simulink model "XTHERM05_reference"  (R2025a)
settings: Solver=daessc  StartTime=0  StopTime=240  MaxStep=1  RelTol=1e-3  AbsTol=1e-3
undefined symbols (not defined in the file): battery_builder_rtmsupport, charge_current_A, charge_step_fraction, charge_step_time_s, coolant_inlet_temperature_K, gcbh, initial_battery_temperature_K
libraries: BatteryPack96S3P_lib x12, fl_lib x8, nesl_utility x5, BatteryCurrentManagement x1, coolingPlateThermal_lib x1
(part 1 of 3)
settings Model: Creator=abirdas  LastModifiedBy=SimuVerity Contributors
settings SolverCC: AutoScaleAbsTol=off
settings SimscapeCC: SimscapeLogType=all  SimscapeLogName=SimlogBattery  SimscapeLogLimitData=off  SimscapeCompileComponentReuse=on
settings ExplorerConfigSet: SimMechanicsOpenEditorOnUpdate=off

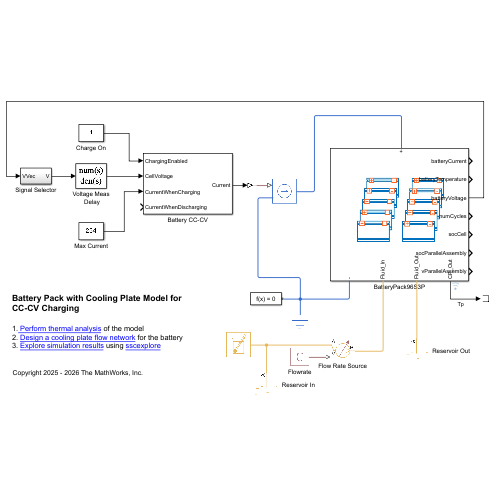
[thumbnail: Simulink's stored preview of the top-level diagram]
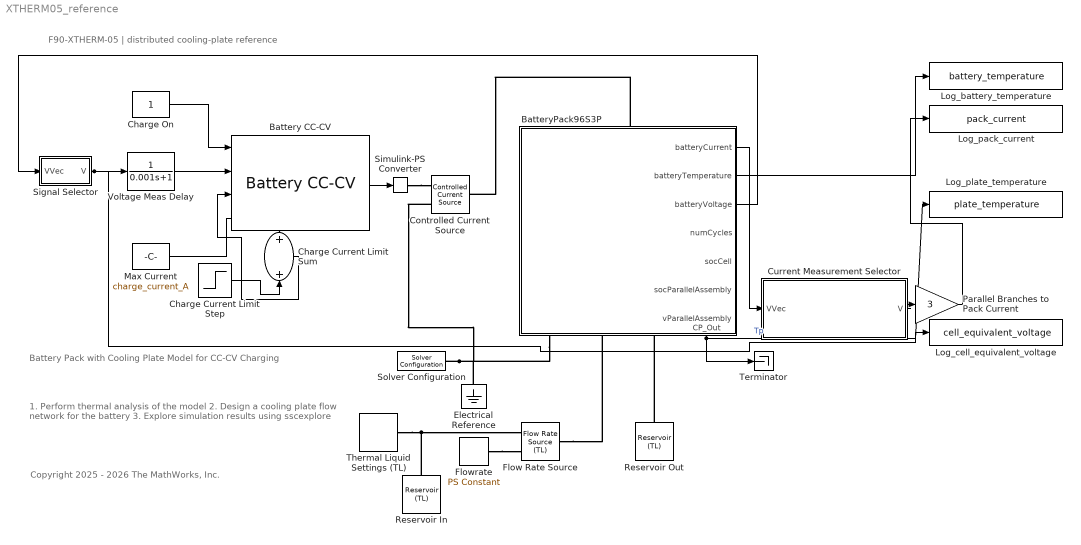
== system XTHERM05_reference ==
  note: 1. Perform thermal analysis of the model
      | 2. Design a cooling plate flow network for the battery
      | 3. Explore simulation results using sscexplore
  note: Copyright 2025 - 2026 The MathWorks, Inc.
  note: Battery Pack with Cooling Plate Model for CC-CV Charging
  note: F90-XTHERM-05 | distributed cooling-plate reference
  Battery CC-CV : BatteryCurrentManagement/Battery CC-CV  MinMaxFlag=off  MaxCellVoltage=max_cell_voltage_V  Kp=100  Ki=1  Kaw=1  Kt=1  Ts=1
      settings: LibrarySourceBlock=batt_sl_lib/Current Management/Battery CC-CV
  BatteryPack96S3P : Subsystem  LoadFcn=battery_builder_rtmsupport('loadfcn',gcbh);
      settings: CopyFcn=battery_builder_rtmsupport('copyfcn',gcbh);  PreCopyFcn=battery_builder_rtmsupport('precopyfcn',gcbh);  PreDeleteFcn=battery_builder_rtmsupport('predeletefcn',gcbh);  PortSchema="{\"entries\":[{\"content\":{\"sides\":[{\"content\":{\"connectorIds\":[\"LConn1\"]},\"type\":\"ConnectorPlacement.EquallySpacedRectSide\",\"uuid\":\"f2fadea4-e63e-44ff-a05d-5cbabbfa18f3\"},{\"content\":{\"connectorIds\":[\"RConn1\",\"RConn2\",\"RConn3\",\"Out1\"],\"side\":\"RIGHT\"},\"type\":\"ConnectorPlacement.EquallySpacedRectSide\",\"uuid\":\"922c0eb8-6335-439b-a096-ecac4f67b25b\"},{\"content\":{\"side\":\"TOP\"},\"type\":\"ConnectorPlacement.EquallySpacedRectSide\",\"uuid\":\"a4ac09f9-1b8b-4b5a-a998-1dae1de64a0b\"},{\"content\":{\"connectorIds\":[\"Out2\",\"Out3\",\"Out4\",\"Out5\",\"Out6\",\"Out7\",\"Out8\"],\"side\":\"BOTTOM\"},\"type\":\"ConnectorPlacement.EquallySpacedRectSide\",\"uuid\":\"64bbb320-f65b-462a-a8f2-7dda0291aa0b\"}]},\"type\":\"ConnectorPlacement.EquallySpacedConnector\",\"uuid\":\"78c9e32e-0392-43f3-93f6-199d4a6b3441\"}],\"packageUris\":[\"http://schema.mathworks.com/mf0/Connector/R2020b\"],\"version\":\"1.0\"}"
      mask Display: image('$imagefile')
  Charge Current Limit Step : Step  Time=charge_step_time_s  After=charge_current_A*charge_step_fraction  SampleTime=0
  Charge Current Limit Sum : Sum
  Charge On : Constant
  Controlled Current Source : fl_lib/Electrical/Electrical Sources/Controlled Current Source
  Current Measurement Selector : Subsystem
  Electrical Reference : fl_lib/Electrical/Electrical Elements/Electrical Reference
  Flow Rate Source : fl_lib/Thermal Liquid/Sources/Flow Rate Source (TL)  source_type=foundation.enum.constant_controlled.controlled  flow_type=foundation.enum.mass_volumetric_flow.volumetric  mass_flow=0 kg/s  volumetric_flow=0 m^3/s  power_spec=foundation.enum.power_spec.isentropic  area=0.01 m^2
      settings: InternalSimscapePortConfiguration="{\"Bottom\":[],\"Left\":[{\"id\":\"A\",\"label\":\"A\",\"type\":\"foundation.thermal_liquid.thermal_liquid\"},{\"id\":\"V\",\"label\":\"V\",\"type\":\"input\"}],\"Right\":[{\"id\":\"B\",\"label\":\"B\",\"type\":\"foundation.thermal_liquid.thermal_liquid\"}],\"Top\":[]}"
  Flowrate : fl_lib/Physical Signals/Sources/PS Constant  constant=coolant_flow_lpm lpm
  Log_battery_temperature : ToWorkspace  VariableName=battery_temperature  SaveFormat=Timeseries  SampleTime=-1
  Log_cell_equivalent_voltage : ToWorkspace  VariableName=cell_equivalent_voltage  SaveFormat=Timeseries  SampleTime=-1
  Log_pack_current : ToWorkspace  VariableName=pack_current  SaveFormat=Timeseries  SampleTime=-1
  Log_plate_temperature : ToWorkspace  VariableName=plate_temperature  SaveFormat=Timeseries  SampleTime=-1
  Max Current : Constant  Value=charge_current_A
  Parallel Branches to Pack Current : Gain  Gain=3
  Reservoir In : fl_lib/Thermal Liquid/Elements/Reservoir (TL)  pressure_spec=foundation.enum.pressure_spec.atmospheric  reservoir_pressure=0.101325 MPa  reservoir_temperature=coolant_inlet_temperature_K K  area=0.01 m^2
  Reservoir Out : fl_lib/Thermal Liquid/Elements/Reservoir (TL)  pressure_spec=foundation.enum.pressure_spec.atmospheric  reservoir_pressure=0.101325 MPa  reservoir_temperature=coolant_inlet_temperature_K K  area=0.01 m^2
  Signal Selector : Subsystem
  Simulink-PS Converter : nesl_utility/Simulink-PS Converter  PhysicalDomain=network_engine_domain  SubClassName=ps_input  LeftPortType=input  RightPortType=output  PseudoPeriodic=off  Frequencies=[]  NoiseDistribution=none  NoiseParameters=[]  Unit=1  AffineConversion=off  FilteringAndDerivatives=provide  SimscapeFilterOrder=1  InputFilterTimeConstant=0.001  UdotUserProvided=0
  Solver Configuration : nesl_utility/Solver Configuration  PhysicalDomain=network_engine_domain  SubClassName=solver  LeftPortType=input  RightPortType=generic  Tones=[]  Harmonics=[]  SimulateNoise=off  Profile=off  UseLocalSampling=off  EnableSwitchedLinearOptims=on  FrequencyDomain=off  UseCCode=off  RelTol=0.001  AbsTol=0.001  MinStep=1e-09  ToWorkspace=off  RevertToSquareIcSolve=off  NumHomotopyIterations=100  PhasorMode=off  PhasorModeNumHarmonics=1  ConsistencySolver=NEWTON_XTOL_AFTER_FTOL  IndexReductionMethod=DerivativeReplacement  DoDC=off  ResidualTolerance=1e-09  ConsistencyTolSource=GLOBAL  ConsistencyAbsTol=0.001  ConsistencyRelTol=0.001  ConsistencyTolFactor=0.001  UseLocalSolver=off  LocalSolverChoice=NE_BACKWARD_EULER_ADVANCER  ResolveIndetEquations=on  FunctionEvalNumThread=1  LocalSolverSampleTime=0.001  DoFixedCost=off  MaxNonlinIter=3  MaxModeIter=2  ComputeImpulses=off  ImpulseIterations=2  LinearAlgebra=auto  LinearAlgebraNumThread=0  EquationFormulation=NE_TIME_EF  DelaysMemoryBudget=1024  AutomaticFiltering=on  FilteringTimeConstant=0.001  PartitionStorageMethod=AS_NEEDED  PartitionMemoryBudget=1024  PartitionMethod=ROBUST  MultibodyUseLocalSolver=off  MultibodyLocalSolverChoice=ODE1  MultibodyLocalSolverSampleTime=0.001
  Terminator : Terminator
  Thermal Liquid Settings (TL) : fl_lib/Thermal Liquid/Utilities/Thermal Liquid Settings (TL)  table_dimensions=foundation.enum.table_dimensions_TL.two_dimensional  T_TLU=[273.1600 : 10 : 373.16]' K  p_TLU=[0.01, 0.1, 5 : 5 : 50] MPa  p_atm=0.101325 MPa  pT_region_flag=foundation.enum.pT_region_TL.min_max  T_min=273.16 K  T_max=373.16 K  p_min=0.01 MPa  p_max=50 MPa  T_min_1D=273.16 K  T_max_1D=373.16 K  p_min_1D=0.01 MPa  p_max_1D=50 MPa  pT_validity_TLU=[1, 1, 1, 1, 1, 1, 1, 1, 1, 1, 1, 1; 1, 1, 1, 1, 1, 1, 1, 1, 1, 1, 1, 1; 1, 1, 1, 1, 1, 1, 1, 1, 1, 1, 1, 1; 1, 1, 1, 1, 1, 1, 1, 1, 1, 1, 1, 1; 1, 1, 1, 1, 1, 1, 1, 1, 1, 1, 1, 1; 0, 1, 1, 1, 1, 1, 1, 1, 1, 1, 1, 1; 0, 1, 1, 1, 1, 1, 1, 1, 1, 1, 1, 1; 0, 1, 1, 1, 1, 1, 1, 1, 1, 1, 1, 1; 0, 1, 1, 1, 1, 1, 1, 1, 1, 1, 1, 1; 0, 1, 1, 1, 1, 1, 1, 1, 1, 1, 1, 1; 0, 0, 1, 1, 1, 1, 1, 1, 1, 1, 1, 1]  properties_range_check=simscape.enum.assert.action.error  rho_parameterization_2D=foundation.enum.rho_parameterization_2D.rho_beta_alpha  rho_parameterization_1D=foundation.enum.rho_parameterization_1D.rho_vector  rho_TLU=[999.7973, 999.8431, 1002.3216, 1004.8218, 1007.293, 1009.7358, 1012.1506, 1014.5379, 1016.8979, 1019.2311, 1021.538, 1023.8188; 999.6579, 999.7009, 1002.0303, 1004.382, 1006.7084, 1009.0101, 1011.2874, 1013.5407, 1015.7703, 1017.9766, 1020.1599, 1022.3206; 998.1632, 998.2045, 1000.4375, 1002.6924, 1004.9239, 1007.1324, 1009.3183, 1011.4819, 1013.6236, 1015.7438, 1017.8428, 1019.921; 995.6057, 995.6458, 997.8186, 1000.0128, 1002.1841, 1004.3332, 1006.4603, 1008.566, 1010.6505, 1012.7144, 1014.758, 1016.7815; 992.1724, 992.2119, 994.3513, 996.5113, 998.6484, 1000.7633, 1002.8563, 1004.928, 1006.9788, 1009.009, 1011.0192, 1013.0097; 988.02, 988.0299, 990.1568, 992.3035, 994.4268, 996.5273, 998.6056, 1000.6622, 1002.6976, 1004.7123, 1006.7067, 1008.6813; 983.18, 983.1901, 985.3217, 987.4721, 989.5983, 991.7008, 993.7803, 995.8374, 997.8726, 999.8864, 1001.8795, 1003.8522; 977.75, 977.7583, 979.9094, 982.0783, 984.2216, 986.34, 988.4343, 990.505, 992.5529, 994.5786, 996.5825, 998.5654; 971.77, 971.7836, 973.9673, 976.1678, 978.3409, 980.4876, 982.6087, 984.7049, 986.7768, 988.8254, 990.8511, 992.8545; 965.26, 965.3023, 967.5311, 969.7753, 971.9901, 974.1764, 976.3354, 978.4676, 980.5741, 982.6556, 984.7129, 986.7465; 958.62, 958.6315, 960.627, 962.9267, 965.1944, 967.4314, 969.6387, 971.8173, 973.9681, 976.0921, 978.19, 980.2628] kg/m^3  beta_TLU=[1.9649, 1.9654, 1.9929, 2.0213, 2.0499, 2.0787, 2.1078, 2.1372, 2.1668, 2.1966, 2.2268, 2.2572; 2.0913, 2.0918, 2.1191, 2.1471, 2.1752, 2.2036, 2.2322, 2.261, 2.2899, 2.3191, 2.3485, 2.3781; 2.1786, 2.1791, 2.2067, 2.235, 2.2634, 2.2919, 2.3206, 2.3494, 2.3784, 2.4075, 2.4367, 2.4661; 2.2332, 2.2337, 2.2619, 2.2908, 2.3197, 2.3487, 2.3778, 2.407, 2.4363, 2.4657, 2.4951, 2.5246; 2.26, 2.2605, 2.2895, 2.3191, 2.3487, 2.3784, 2.4081, 2.4378, 2.4675, 2.4973, 2.5272, 2.5571; 2.2638, 2.2638, 2.2936, 2.324, 2.3544, 2.3848, 2.4151, 2.4455, 2.4758, 2.5062, 2.5365, 2.5669; 2.2472, 2.2472, 2.2779, 2.3092, 2.3403, 2.3715, 2.4025, 2.4336, 2.4646, 2.4955, 2.5264, 2.5573; 2.214, 2.214, 2.2455, 2.2776, 2.3096, 2.3415, 2.3733, 2.405, 2.4367, 2.4683, 2.4998, 2.5313; 2.1668, 2.1668, 2.1992, 2.2321, 2.2649, 2.2976, 2.3301, 2.3626, 2.3949, 2.4272, 2.4593, 2.4914; 2.1081, 2.1081, 2.1413, 2.175, 2.2086, 2.2421, 2.2754, 2.3085, 2.3415, 2.3744, 2.4072, 2.4399; 2.0494, 2.0494, 2.0739, 2.1084, 2.1428, 2.177, 2.211, 2.2449, 2.2786, 2.3121, 2.3455, 2.3788] GPa  alpha_TLU=1e-4 * [-.679, -.676, -.49, -.307, -.13, .041, .206, .365, .519, .668, .811, .949; .878, .881, .998, 1.114, 1.227, 1.337, 1.445, 1.549, 1.651, 1.75, 1.846, 1.939; 2.068, 2.069, 2.141, 2.213, 2.283, 2.352, 2.42, 2.486, 2.551, 2.614, 2.676, 2.736; 3.034, 3.035, 3.074, 3.113, 3.152, 3.191, 3.229, 3.267, 3.305, 3.341, 3.377, 3.413; 3.855, 3.856, 3.87, 3.884, 3.899, 3.914, 3.93, 3.946, 3.961, 3.977, 3.993, 4.009; 4.578, 4.578, 4.572, 4.566, 4.562, 4.558, 4.555, 4.552, 4.55, 4.549, 4.548, 4.547; 5.233, 5.233, 5.209, 5.186, 5.165, 5.144, 5.125, 5.107, 5.09, 5.074, 5.059, 5.045; 5.84, 5.84, 5.801, 5.762, 5.725, 5.691, 5.657, 5.625, 5.595, 5.566, 5.538, 5.512; 6.414, 6.414, 6.36, 6.307, 6.256, 6.208, 6.161, 6.117, 6.074, 6.033, 5.994, 5.956; 6.967, 6.967, 6.898, 6.831, 6.766, 6.705, 6.646, 6.589, 6.535, 6.482, 6.432, 6.384; 7.519, 7.519, 7.423, 7.342, 7.264, 7.189, 7.118, 7.049, 6.983, 6.92, 6.859, 6.8] 1/K  rho_TLU_2=[999.7973, 999.8431, 1002.3216, 1004.8218, 1007.293, 1009.7358, 1012.1506, 1014.5379, 1016.8979, 1019.2311, 1021.538, 1023.8188; 999.6579, 999.7009, 1002.0303, 1004.382, 1006.7084, 1009.0101, 1011.2874, 1013.5407, 1015.7703, 1017.9766, 1020.1599, 1022.3206; 998.1632, 998.2045, 1000.4375, 1002.6924, 1004.9239, 1007.1324, 1009.3183, 1011.4819, 1013.6236, 1015.7438, 1017.8428, 1019.921; 995.6057, 995.6458, 997.81864, 1000.0128, 1002.1841, 1004.3332, 1006.4603, 1008.566, 1010.6505, 1012.7144, 1014.758, 1016.7815; 992.1724, 992.2119, 994.3513, 996.5113, 998.6484, 1000.7633, 1002.8563, 1004.928, 1006.9788, 1009.009, 1011.0192, 1013.0097; 988.02, 988.0299, 990.1568, 992.3035, 994.4268, 996.5273, 998.6056, 1000.6622, 1002.6976, 1004.7123, 1006.7067, 1008.6813; 983.18, 983.1901, 985.3217, 987.4721, 989.5983, 991.7008, 993.7803, 995.8374, 997.8726, 999.8864, 1001.8795, 1003.8522; 977.75, 977.7583, 979.9094, 982.0783, 984.2216, 986.34, 988.4343, 990.505, 992.5529, 994.5786, 996.5825, 998.5654; 971.77, 971.7836, 973.9673, 976.1678, 978.3409, 980.4876, 982.6087, 984.7049, 986.7768, 988.8254, 990.8511, 992.8545; 965.26, 965.3023, 967.5311, 969.7753, 971.9901, 974.1764, 976.3354, 978.4676, 980.5741, 982.6556, 984.7129, 986.7465; 958.62, 958.6315, 960.627, 962.9267, 965.1944, 967.4314, 969.6387, 971.8173, 973.9681, 976.0921, 978.19, 980.2628] kg/m^3  rho_ref_3=998.21 kg/m^3  T_ref_3=293.16 K  p_ref_3=0.101325 MPa  beta_const_3=2.1791 GPa  alpha_const_3=2.0691e-4 1/K  rho_TLU_4=[999.84; 999.7; 998.2; 995.65; 992.21; 988.03; 983.19; 977.76; 971.78; 965.3; 958.8] kg/m^3  beta_const_4=2.1791 GPa  p_ref_4=0.101325 MPa  rho_ref_5=998.21 kg/m^3  T_ref_5=293.16 K  p_ref_5=0.101325 MPa  beta_const_5=2.1791 GPa  alpha_const_5=2.0691e-4 1/K  u_parameterization_2D=foundation.enum.u_parameterization_2D.u_cp  u_parameterization_1D=foundation.enum.u_parameterization_1D.u  u_TLU=[.0002, .0018, .086, .1588, .219, .267, .3034, .3288, .3436, .3483, .3435, .3294; 42.062, 42.06, 41.935, 41.804, 41.668, 41.527, 41.382, 41.233, 41.081, 40.924, 40.763, 40.599; 83.953, 83.948, 83.651, 83.349, 83.049, 82.749, 82.451, 82.153, 81.856, 81.56, 81.265, 80.971; 125.77, 125.76, 125.31, 124.86, 124.41, 123.97, 123.53, 123.1, 122.68, 122.25, 121.84, 121.42; 167.57, 167.56, 166.96, 166.37, 165.79, 165.21, 164.65, 164.09, 163.54, 163, 162.46, 161.94; 209.36, 209.36, 208.63, 207.9, 207.19, 206.48, 205.79, 205.11, 204.45, 203.79, 203.14, 202.5; 251.19, 251.19, 250.33, 249.47, 248.62, 247.79, 246.98, 246.18, 245.39, 244.62, 243.86, 243.12; 293.06, 293.06, 292.07, 291.07, 290.1, 289.14, 288.2, 287.28, 286.38, 285.49, 284.62, 283.77; 334.99, 334.99, 333.86, 332.73, 331.63, 330.54, 329.48, 328.44, 327.41, 326.41, 325.43, 324.46; 377, 377, 375.73, 374.46, 373.22, 372, 370.81, 369.64, 368.5, 367.38, 366.27, 365.19; 419.01, 419.01, 417.69, 416.27, 414.89, 413.54, 412.21, 410.91, 409.64, 408.4, 407.17, 405.98] kJ/kg  cp_TLU=[4.2199, 4.2194, 4.1957, 4.1726, 4.1508, 4.13, 4.1103, 4.0916, 4.0738, 4.0569, 4.0408, 4.0254; 4.1955, 4.1951, 4.1769, 4.1592, 4.1422, 4.1259, 4.1103, 4.0954, 4.0812, 4.0676, 4.0545, 4.0421; 4.1843, 4.184, 4.169, 4.1543, 4.1401, 4.1264, 4.1133, 4.1007, 4.0885, 4.0768, 4.0656, 4.0548; 4.1801, 4.1798, 4.1667, 4.1538, 4.1413, 4.1293, 4.1177, 4.1064, 4.0956, 4.0851, 4.075, 4.0653; 4.1796, 4.1794, 4.1675, 4.1558, 4.1444, 4.1334, 4.1227, 4.1123, 4.1023, 4.0926, 4.0832, 4.0741; 4.1813, 4.1813, 4.1702, 4.1592, 4.1484, 4.138, 4.1279, 4.1181, 4.1086, 4.0993, 4.0903, 4.0816; 4.185, 4.185, 4.1742, 4.1636, 4.1532, 4.1432, 4.1334, 4.1239, 4.1146, 4.1056, 4.0969, 4.0884; 4.1901, 4.1901, 4.1795, 4.169, 4.1588, 4.1489, 4.1393, 4.1299, 4.1207, 4.1118, 4.1032, 4.0947; 4.1968, 4.1968, 4.1862, 4.1757, 4.1655, 4.1555, 4.1458, 4.1364, 4.1273, 4.1183, 4.1096, 4.1012; 4.2052, 4.2052, 4.1944, 4.1837, 4.1733, 4.1632, 4.1534, 4.1438, 4.1345, 4.1255, 4.1166, 4.108; 4.2136, 4.2136, 4.2045, 4.1935, 4.1828, 4.1724, 4.1623, 4.1524, 4.1429, 4.1335, 4.1245, 4.1157] kJ/(K*kg)  u_TLU_2=[.0002, .0018, .086, .1588, .219, .267, .3034, .3288, .3436, .3483, .3435, .3294; 42.062, 42.06, 41.935, 41.804, 41.668, 41.527, 41.382, 41.233, 41.081, 40.924, 40.763, 40.599; 83.953, 83.948, 83.651, 83.349, 83.049, 82.749, 82.451, 82.153, 81.856, 81.56, 81.265, 80.971; 125.77, 125.76, 125.31, 124.86, 124.41, 123.97, 123.53, 123.1, 122.68, 122.25, 121.84, 121.42; 167.57, 167.56, 166.96, 166.37, 165.79, 165.21, 164.65, 164.09, 163.54, 163, 162.46, 161.94; 209.36, 209.36, 208.63, 207.9, 207.19, 206.48, 205.79, 205.11, 204.45, 203.79, 203.14, 202.5; 251.19, 251.19, 250.33, 249.47, 248.62, 247.79, 246.98, 246.18, 245.39, 244.62, 243.86, 243.12; 293.06, 293.06, 292.07, 291.07, 290.1, 289.14, 288.2, 287.28, 286.38, 285.49, 284.62, 283.77; 334.99, 334.99, 333.86, 332.73, 331.63, 330.54, 329.48, 328.44, 327.41, 326.41, 325.43, 324.46; 377, 377, 375.73, 374.46, 373.22, 372, 370.81, 369.64, 368.5, 367.38, 366.27, 365.19; 419.01, 419.01, 417.69, 416.27, 414.89, 413.54, 412.21, 410.91, 409.64, 408.4, 407.17, 405.98] kJ/kg  cp_TLU_3=[4.2199, 4.2194, 4.1957, 4.1726, 4.1508, 4.13, 4.1103, 4.0916, 4.0738, 4.0569, 4.0408, 4.0254; 4.1955, 4.1951, 4.1769, 4.1592, 4.1422, 4.1259, 4.1103, 4.0954, 4.0812, 4.0676, 4.0545, 4.0421; 4.1843, 4.184, 4.169, 4.1543, 4.1401, 4.1264, 4.1133, 4.1007, 4.0885, 4.0768, 4.0656, 4.0548; 4.1801, 4.1798, 4.1667, 4.1538, 4.1413, 4.1293, 4.1177, 4.1064, 4.0956, 4.0851, 4.075, 4.0653; 4.1796, 4.1794, 4.1675, 4.1558, 4.1444, 4.1334, 4.1227, 4.1123, 4.1023, 4.0926, 4.0832, 4.0741; 4.1813, 4.1813, 4.1702, 4.1592, 4.1484, 4.138, 4.1279, 4.1181, 4.1086, 4.0993, 4.0903, 4.0816; 4.185, 4.185, 4.1742, 4.1636, 4.1532, 4.1432, 4.1334, 4.1239, 4.1146, 4.1056, 4.0969, 4.0884; 4.1901, 4.1901, 4.1795, 4.169, 4.1588, 4.1489, 4.1393, 4.1299, 4.1207, 4.1118, 4.1032, 4.0947; 4.1968, 4.1968, 4.1862, 4.1757, 4.1655, 4.1555, 4.1458, 4.1364, 4.1273, 4.1183, 4.1096, 4.1012; 4.2052, 4.2052, 4.1944, 4.1837, 4.1733, 4.1632, 4.1534, 4.1438, 4.1345, 4.1255, 4.1166, 4.108; 4.2136, 4.2136, 4.2045, 4.1935, 4.1828, 4.1724, 4.1623, 4.1524, 4.1429, 4.1335, 4.1245, 4.1157] kJ/(K*kg)  u_TLU_4=[.0018; 42.06; 83.948; 125.76; 167.56; 209.36; 251.19; 293.06; 334.99; 377; 418.01] kJ/kg  cp_TLU_5=[4.2199; 4.1955; 4.1843; 4.1801; 4.1796; 4.1813; 4.185; 4.1901; 4.1968; 4.2052; 4.2136] kJ/(K*kg)  nu_TLU=[1.7917, 1.7914, 1.7763, 1.7615, 1.7473, 1.7338, 1.7208, 1.7085, 1.6967, 1.6854, 1.6747, 1.6645; 1.3061, 1.3059, 1.2986, 1.2914, 1.2845, 1.2779, 1.2716, 1.2656, 1.2598, 1.2543, 1.2491, 1.2441; 1.0032, 1.0032, .9995, .9959, .9924, .9891, .9859, .9829, .9801, .9774, .9748, .9724; .8006, .8005, .7987, .797, .7953, .7937, .7922, .7908, .7894, .7881, .787, .7859; .6577, .6577, .657, .6562, .6555, .6548, .6543, .6537, .6532, .6528, .6523, .652; .553, .553, .5529, .5527, .5526, .5525, .5524, .5524, .5524, .5524, .5524, .5525; .4739, .4739, .4741, .4743, .4745, .4747, .475, .4753, .4755, .4758, .4762, .4765; .4127, .4127, .4131, .4135, .4139, .4143, .4148, .4152, .4157, .4162, .4167, .4172; .3643, .3643, .3648, .3654, .3659, .3665, .367, .3676, .3682, .3688, .3694, .37; .3254, .3254, .3261, .3267, .3273, .328, .3286, .3293, .3299, .3306, .3312, .3319; .2866, .2866, .2945, .2952, .2959, .2965, .2972, .2979, .2986, .2993, .3, .3007] mm^2/s  nu_TLU_2=[1.7917; 1.3061; 1.0032; .8006; .6577; .553; .4739; .4127; .3643; .3254; .2866] mm^2/s  k_TLU=[561.04, 561.09, 563.8, 566.56, 569.32, 572.08, 574.82, 577.54, 580.24, 582.92, 585.57, 588.18; 580.02, 580.07, 582.45, 584.88, 587.32, 589.75, 592.18, 594.61, 597.02, 599.42, 601.8, 604.16; 598.44, 598.48, 600.73, 603.03, 605.33, 607.64, 609.94, 612.24, 614.54, 616.82, 619.1, 621.36; 615.48, 615.52, 617.73, 620, 622.26, 624.54, 626.81, 629.07, 631.34, 633.6, 635.85, 638.09; 630.6, 630.64, 632.87, 635.15, 637.44, 639.72, 642.01, 644.29, 646.57, 648.84, 651.11, 653.36; 643.61, 643.61, 645.88, 648.21, 650.53, 652.86, 655.18, 657.51, 659.82, 662.14, 664.44, 666.74; 654.39, 654.39, 656.73, 659.12, 661.5, 663.89, 666.27, 668.65, 671.02, 673.38, 675.74, 678.09; 663.13, 663.13, 665.54, 668, 670.46, 672.91, 675.36, 677.8, 680.24, 682.67, 685.09, 687.5; 670.02, 670.02, 672.51, 675.05, 677.59, 680.12, 682.64, 685.16, 687.67, 690.17, 692.66, 695.14; 675.27, 675.27, 677.85, 680.48, 683.11, 685.73, 688.34, 690.94, 693.53, 696.11, 698.68, 701.24; 680.52, 680.52, 681.77, 684.5, 687.22, 689.94, 692.64, 695.34, 698.02, 700.69, 703.35, 706] mW/(K*m)  k_TLU_2=[561.04; 580.02; 598.44; 615.48; 630.6; 643.61; 654.39; 663.13; 670.02; 675.27; 680.52] mW/(K*m)
  Voltage Meas Delay : TransferFcn  Denominator=[0.001 1]
  wires:
  Signal Selector/1(V) -> Voltage Meas Delay/1, Log_cell_equivalent_voltage/1
  Battery CC-CV/1 -> Simulink-PS Converter/1
  Voltage Meas Delay/1 -> Battery CC-CV/2
  Charge On/1 -> Battery CC-CV/1
  BatteryPack96S3P/1(CP_Out) -> Terminator/1, Log_plate_temperature/1  "Tp"
  BatteryPack96S3P/4(batteryVoltage) -> Signal Selector/1(VVec)
  Max Current/1 -> Charge Current Limit Sum/1
  Charge Current Limit Step/1 -> Charge Current Limit Sum/2
  Charge Current Limit Sum/1 -> Battery CC-CV/3
  BatteryPack96S3P/3(batteryTemperature) -> Log_battery_temperature/1
  BatteryPack96S3P/2(batteryCurrent) -> Current Measurement Selector/1(VVec)
  Current Measurement Selector/1(V) -> Parallel Branches to Pack Current/1
  Parallel Branches to Pack Current/1 -> Log_pack_current/1
  connections:
  Thermal Liquid Settings (TL)/RConn1 -- Flow Rate Source/LConn1 -- Reservoir In/LConn1
  Solver Configuration/RConn1 -- BatteryPack96S3P/RConn1 -- Electrical Reference/LConn1 -- Controlled Current Source/RConn2
  Simulink-PS Converter/RConn1 -- Controlled Current Source/RConn1
  BatteryPack96S3P/LConn1 -- Controlled Current Source/LConn1
  Flowrate/RConn1 -- Flow Rate Source/LConn2
  Reservoir Out/LConn1 -- BatteryPack96S3P/RConn3
  Flow Rate Source/RConn1 -- BatteryPack96S3P/RConn2

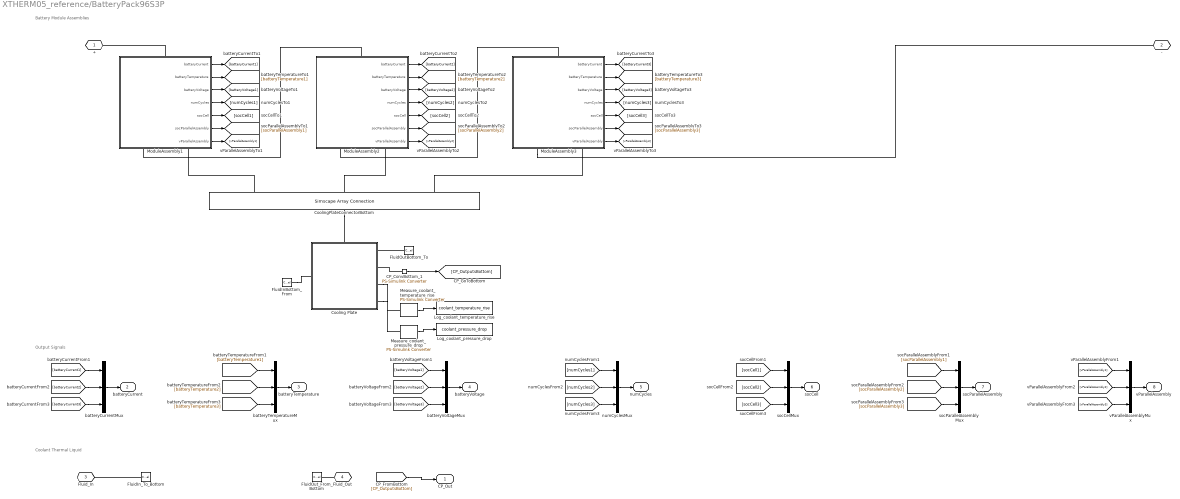
== system XTHERM05_reference/BatteryPack96S3P ==
  note: Battery Module Assemblies
  note: Output Signals
  note: Coolant Thermal Liquid
  CP_ConvBottom_1 : nesl_utility/PS-Simulink Converter  PhysicalDomain=network_engine_domain  SubClassName=ps_output  LeftPortType=input  RightPortType=output  PseudoPeriodic=off  Frequencies=[]  VectorFormat=inherit  Unit=inherit  AffineConversion=off
  Cooling Plate : Subsystem  AncestorBlock=BatteryCoolingPlate_lib/Cooling Plate  mask{numBattThermalNodes=24, dimensionThermalNodes=[0.36 0.143;0.36 0.143;0.36 0.143;0.36 0.143;0.36 0.143;0.36 0.143;0.36 0.143;0.36 0.143;0.36 0.143;0.36 0.143;0.36 0.143;0.36 0.143;0.36 0.143;0.36 0.143;0.36 0.143;0.36 0.143;0.36 0.143;0.36 0.143;0.36 0.143;0.36 0.143;0.36 0.143;0.36 0.143;0.36 0.143;0.36 0.143], locationThermalNodes=[0.18 0.0715;0.18 0.2195;0.18 0.3725;0.18 0.5205;0.18 0.6735;0.18 0.821500000000001;0.18 0.9745;0.18 1.1225;0.55 0.0715;0.55 0.2195;0.55 0.3725;0.55 0.5205;0.55 0.6735;0.55 0.821500000000001;0.55 0.9745;0.55 1.1225;0.92 0.0715;0.92 0.2195;0.92 0.3725;0.92 0.5205;0.92 0.6735;0.92 0.821500000000001;0.92 0.9745;0.92 1.1225], plateDimX=3, plateDimY=8, thkPlate=0.008, thCondPlate=20, rhoPlate=2700, cpPlate=447, initTempPlate=coolant_inlet_temperature_K}
      mask prompts: numBattThermalNodes "Number of battery thermal nodes"; dimensionThermalNodes "Dimension of battery thermal nodes (m)"; locationThermalNodes "Coordinates of battery thermal nodes (m)"; plateDimX "Number of partitions in X direction"; plateDimY "Number of partitions in Y direction"; thkPlate "Thickness of cooling plate (m)"; thCondPlate "Thermal conductivity of cooling plate material (W/(K*m))"; rhoPlate "Density of cooling plate material (kg/m^3)"; cpPlate "Specific heat of cooling plate material (J/(K*kg))"; initTempPlate "Initial temperature of cooling plate and coolant (K)"
      settings: PortSchema="{\"entries\":[{\"content\":{\"sides\":[{\"content\":{\"connectorIds\":[\"LConn1\"]},\"type\":\"ConnectorPlacement.EquallySpacedRectSide\",\"uuid\":\"61d09505-4787-4116-9e09-ef2c1cc64727\"},{\"content\":{\"connectorIds\":[\"RConn1\",\"RConn2\",\"RConn3\",\"RConn4\"],\"side\":\"RIGHT\"},\"type\":\"ConnectorPlacement.EquallySpacedRectSide\",\"uuid\":\"8778701f-9770-4a80-b014-3c62d1dc85cd\"},{\"content\":{\"connectorIds\":[\"LConn2\"],\"side\":\"TOP\"},\"type\":\"ConnectorPlacement.EquallySpacedRectSide\",\"uuid\":\"7fe4cd3b-1140-4af6-8c89-d00184ab11c4\"}]},\"type\":\"ConnectorPlacement.EquallySpacedConnector\",\"uuid\":\"d686b711-433f-43c2-a2f7-d5d5927dd9dd\"}],\"packageUris\":[\"http://schema.mathworks.com/mf0/Connector/R2020b\"],\"version\":\"1.0\"}"
      mask DialogControl MainGroup Prompt: Settings
      mask DialogControl InterfacePanel Prompt: Interface
      mask DialogControl MaterialPanel Prompt: Plate Material
      mask Display: image('CoolingPlateMaskIcon.png')
  CoolingPlateConnectorBottom : SimscapeArrayConnection  Domain=foundation.thermal.thermal  Mode=Sized Elements
  FluidInBottom_From : ConnectionLabel  Label=FluidIn_To_Bottom
  FluidIn_To_Bottom : ConnectionLabel  Label=FluidIn_To_Bottom
  FluidOutBottom_To : ConnectionLabel  Label=FluidOut_From_Bottom
  FluidOut_From_Bottom : ConnectionLabel  Label=FluidOut_From_Bottom
  Log_coolant_pressure_drop : ToWorkspace  VariableName=coolant_pressure_drop  SaveFormat=Timeseries  SampleTime=-1
  Log_coolant_temperature_rise : ToWorkspace  VariableName=coolant_temperature_rise  SaveFormat=Timeseries  SampleTime=-1
  Measure_coolant_pressure_drop : nesl_utility/PS-Simulink Converter  PhysicalDomain=network_engine_domain  SubClassName=ps_output  LeftPortType=input  RightPortType=output  PseudoPeriodic=off  Frequencies=[]  VectorFormat=inherit  Unit=bar  AffineConversion=off
  Measure_coolant_temperature_rise : nesl_utility/PS-Simulink Converter  PhysicalDomain=network_engine_domain  SubClassName=ps_output  LeftPortType=input  RightPortType=output  PseudoPeriodic=off  Frequencies=[]  VectorFormat=inherit  Unit=K  AffineConversion=off
  ModuleAssembly1 : Subsystem  LoadFcn=battery_builder_rtmsupport('loadfcn',gcbh);
      settings: CopyFcn=battery_builder_rtmsupport('copyfcn',gcbh);  PreCopyFcn=battery_builder_rtmsupport('precopyfcn',gcbh);  PreDeleteFcn=battery_builder_rtmsupport('predeletefcn',gcbh);  PortSchema="{\"entries\":[{\"content\":{\"sides\":[{\"content\":{\"connectorIds\":[\"LConn1\"]},\"type\":\"ConnectorPlacement.EquallySpacedRectSide\",\"uuid\":\"503de65f-eb03-4dca-ae24-61c84f956962\"},{\"content\":{\"connectorIds\":[\"RConn1\",\"RConn2\"],\"side\":\"RIGHT\"},\"type\":\"ConnectorPlacement.EquallySpacedRectSide\",\"uuid\":\"ec12e430-573b-4590-abb2-9abeb9cda924\"},{\"content\":{\"side\":\"TOP\"},\"type\":\"ConnectorPlacement.EquallySpacedRectSide\",\"uuid\":\"53716a75-1aaa-4105-9001-c0fcf257a33a\"},{\"content\":{\"connectorIds\":[\"Out1\",\"Out2\",\"Out3\",\"Out4\",\"Out5\",\"Out6\",\"Out7\"],\"side\":\"BOTTOM\"},\"type\":\"ConnectorPlacement.EquallySpacedRectSide\",\"uuid\":\"dbdc6f0e-c03f-471b-88ec-220339ff01d4\"}]},\"type\":\"ConnectorPlacement.EquallySpacedConnector\",\"uuid\":\"3a01d345-c1d7-4c9f-9700-ee1665611d8c\"}],\"packageUris\":[\"http://schema.mathworks.com/mf0/Connector/R2020b\"],\"version\":\"1.0\"}"
      mask Display: image('moduleAssembly_1.JPG');
  ModuleAssembly2 : Subsystem  LoadFcn=battery_builder_rtmsupport('loadfcn',gcbh);
      settings: CopyFcn=battery_builder_rtmsupport('copyfcn',gcbh);  PreCopyFcn=battery_builder_rtmsupport('precopyfcn',gcbh);  PreDeleteFcn=battery_builder_rtmsupport('predeletefcn',gcbh);  PortSchema="{\"entries\":[{\"content\":{\"sides\":[{\"content\":{\"connectorIds\":[\"LConn1\"]},\"type\":\"ConnectorPlacement.EquallySpacedRectSide\",\"uuid\":\"503de65f-eb03-4dca-ae24-61c84f956962\"},{\"content\":{\"connectorIds\":[\"RConn1\",\"RConn2\"],\"side\":\"RIGHT\"},\"type\":\"ConnectorPlacement.EquallySpacedRectSide\",\"uuid\":\"ec12e430-573b-4590-abb2-9abeb9cda924\"},{\"content\":{\"side\":\"TOP\"},\"type\":\"ConnectorPlacement.EquallySpacedRectSide\",\"uuid\":\"53716a75-1aaa-4105-9001-c0fcf257a33a\"},{\"content\":{\"connectorIds\":[\"Out1\",\"Out2\",\"Out3\",\"Out4\",\"Out5\",\"Out6\",\"Out7\"],\"side\":\"BOTTOM\"},\"type\":\"ConnectorPlacement.EquallySpacedRectSide\",\"uuid\":\"dbdc6f0e-c03f-471b-88ec-220339ff01d4\"}]},\"type\":\"ConnectorPlacement.EquallySpacedConnector\",\"uuid\":\"3a01d345-c1d7-4c9f-9700-ee1665611d8c\"}],\"packageUris\":[\"http://schema.mathworks.com/mf0/Connector/R2020b\"],\"version\":\"1.0\"}"
      mask Display: image('moduleAssembly_2.JPG');
  ModuleAssembly3 : Subsystem  LoadFcn=battery_builder_rtmsupport('loadfcn',gcbh);
      settings: CopyFcn=battery_builder_rtmsupport('copyfcn',gcbh);  PreCopyFcn=battery_builder_rtmsupport('precopyfcn',gcbh);  PreDeleteFcn=battery_builder_rtmsupport('predeletefcn',gcbh);  PortSchema="{\"entries\":[{\"content\":{\"sides\":[{\"content\":{\"connectorIds\":[\"LConn1\"]},\"type\":\"ConnectorPlacement.EquallySpacedRectSide\",\"uuid\":\"503de65f-eb03-4dca-ae24-61c84f956962\"},{\"content\":{\"connectorIds\":[\"RConn1\",\"RConn2\"],\"side\":\"RIGHT\"},\"type\":\"ConnectorPlacement.EquallySpacedRectSide\",\"uuid\":\"ec12e430-573b-4590-abb2-9abeb9cda924\"},{\"content\":{\"side\":\"TOP\"},\"type\":\"ConnectorPlacement.EquallySpacedRectSide\",\"uuid\":\"53716a75-1aaa-4105-9001-c0fcf257a33a\"},{\"content\":{\"connectorIds\":[\"Out1\",\"Out2\",\"Out3\",\"Out4\",\"Out5\",\"Out6\",\"Out7\"],\"side\":\"BOTTOM\"},\"type\":\"ConnectorPlacement.EquallySpacedRectSide\",\"uuid\":\"dbdc6f0e-c03f-471b-88ec-220339ff01d4\"}]},\"type\":\"ConnectorPlacement.EquallySpacedConnector\",\"uuid\":\"3a01d345-c1d7-4c9f-9700-ee1665611d8c\"}],\"packageUris\":[\"http://schema.mathworks.com/mf0/Connector/R2020b\"],\"version\":\"1.0\"}"
      mask Display: image('moduleAssembly_3.JPG');
  batteryCurrentMux : Mux  Inputs=3
  batteryTemperatureMux : Mux  Inputs=3
  batteryVoltageMux : Mux  Inputs=3
  numCyclesMux : Mux  Inputs=3
  socCellMux : Mux  Inputs=3
  socParallelAssemblyMux : Mux  Inputs=3
  vParallelAssemblyMux : Mux  Inputs=3
  + : PMIOPort  Side=Left
  - : PMIOPort  Port=2  Side=Right
  Fluid_In : PMIOPort  Port=3  Side=Right  ConnectionType=Connection: foundation.thermal_liquid.thermal_liquid
  Fluid_Out : PMIOPort  Port=4  Side=Right  ConnectionType=Connection: foundation.thermal_liquid.thermal_liquid
  CP_Out : Outport
  batteryCurrent : Outport  Port=2
  batteryTemperature : Outport  Port=3
  batteryVoltage : Outport  Port=4
  numCycles : Outport  Port=5
  socCell : Outport  Port=6
  socParallelAssembly : Outport  Port=7
  vParallelAssembly : Outport  Port=8
  wires:
  ModuleAssembly1/1(batteryCurrent) -> [batteryCurrent1]
  batteryCurrentMux/1 -> batteryCurrent/1
  [batteryCurrent1] -> batteryCurrentMux/1
  ModuleAssembly1/2(batteryTemperature) -> [batteryTemperature1]
  batteryTemperatureMux/1 -> batteryTemperature/1
  [batteryTemperature1] -> batteryTemperatureMux/1
  ModuleAssembly1/3(batteryVoltage) -> [batteryVoltage1]
  batteryVoltageMux/1 -> batteryVoltage/1
  [batteryVoltage1] -> batteryVoltageMux/1
  ModuleAssembly1/4(numCycles) -> [numCycles1]
  numCyclesMux/1 -> numCycles/1
  [numCycles1] -> numCyclesMux/1
  ModuleAssembly1/5(socCell) -> [socCell1]
  socCellMux/1 -> socCell/1
  [socCell1] -> socCellMux/1
  ModuleAssembly1/6(socParallelAssembly) -> [socParallelAssembly1]
  socParallelAssemblyMux/1 -> socParallelAssembly/1
  [socParallelAssembly1] -> socParallelAssemblyMux/1
  ModuleAssembly1/7(vParallelAssembly) -> [vParallelAssembly1]
  vParallelAssemblyMux/1 -> vParallelAssembly/1
  [vParallelAssembly1] -> vParallelAssemblyMux/1
  ModuleAssembly2/1(batteryCurrent) -> [batteryCurrent2]
  [batteryCurrent2] -> batteryCurrentMux/2
  ModuleAssembly2/2(batteryTemperature) -> [batteryTemperature2]
  [batteryTemperature2] -> batteryTemperatureMux/2
  ModuleAssembly2/3(batteryVoltage) -> [batteryVoltage2]
  [batteryVoltage2] -> batteryVoltageMux/2
  ModuleAssembly2/4(numCycles) -> [numCycles2]
  [numCycles2] -> numCyclesMux/2
  ModuleAssembly2/5(socCell) -> [socCell2]
  [socCell2] -> socCellMux/2
  ModuleAssembly2/6(socParallelAssembly) -> [socParallelAssembly2]
  [socParallelAssembly2] -> socParallelAssemblyMux/2
  ModuleAssembly2/7(vParallelAssembly) -> [vParallelAssembly2]
  [vParallelAssembly2] -> vParallelAssemblyMux/2
  ModuleAssembly3/1(batteryCurrent) -> [batteryCurrent3]
  [batteryCurrent3] -> batteryCurrentMux/3
  ModuleAssembly3/2(batteryTemperature) -> [batteryTemperature3]
  [batteryTemperature3] -> batteryTemperatureMux/3
  ModuleAssembly3/3(batteryVoltage) -> [batteryVoltage3]
  [batteryVoltage3] -> batteryVoltageMux/3
  ModuleAssembly3/4(numCycles) -> [numCycles3]
  [numCycles3] -> numCyclesMux/3
  ModuleAssembly3/5(socCell) -> [socCell3]
  [socCell3] -> socCellMux/3
  ModuleAssembly3/6(socParallelAssembly) -> [socParallelAssembly3]
  [socParallelAssembly3] -> socParallelAssemblyMux/3
  ModuleAssembly3/7(vParallelAssembly) -> [vParallelAssembly3]
  [vParallelAssembly3] -> vParallelAssemblyMux/3
  CP_ConvBottom_1/1 -> [CP_OutputsBottom]
  [CP_OutputsBottom] -> CP_Out/1
  Measure_coolant_temperature_rise/1 -> Log_coolant_temperature_rise/1
  Measure_coolant_pressure_drop/1 -> Log_coolant_pressure_drop/1
  connections:
  ModuleAssembly2/LConn1 -- ModuleAssembly1/RConn1
  ModuleAssembly3/LConn1 -- ModuleAssembly2/RConn1
  ModuleAssembly1/LConn1 -- +/RConn1
  ModuleAssembly3/RConn1 -- -/RConn1
  CoolingPlateConnectorBottom/LConn1 -- ModuleAssembly1/RConn2
  CoolingPlateConnectorBottom/LConn2 -- ModuleAssembly2/RConn2
  CoolingPlateConnectorBottom/LConn3 -- ModuleAssembly3/RConn2
  CoolingPlateConnectorBottom/RConn1 -- Cooling Plate/LConn2
  FluidIn_To_Bottom/LConn1 -- Fluid_In/RConn1
  Fluid_Out/RConn1 -- FluidOut_From_Bottom/LConn1
  FluidInBottom_From/LConn1 -- Cooling Plate/LConn1
  FluidOutBottom_To/LConn1 -- Cooling Plate/RConn1
  CP_ConvBottom_1/LConn1 -- Cooling Plate/RConn2
  Cooling Plate/RConn3 -- Measure_coolant_temperature_rise/LConn1
  Cooling Plate/RConn4 -- Measure_coolant_pressure_drop/LConn1

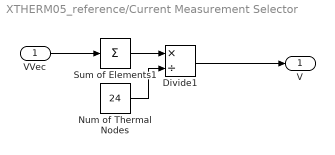
== system XTHERM05_reference/Current Measurement Selector ==
  VVec : Inport
  Divide1 : Product  Inputs=*/
  Num of Thermal Nodes : Constant  Value=24
  Sum of Elements1 : Sum  Inputs=+
  V : Outport
  wires:
  Num of Thermal Nodes/1 -> Divide1/2
  Sum of Elements1/1 -> Divide1/1
  Divide1/1 -> V/1
  VVec/1 -> Sum of Elements1/1

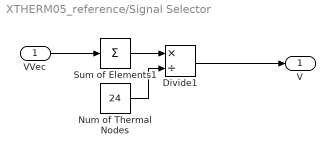
== system XTHERM05_reference/Signal Selector ==
  VVec : Inport
  Divide1 : Product  Inputs=*/
  Num of Thermal Nodes : Constant  Value=24
  Sum of Elements1 : Sum  Inputs=+
  V : Outport
  wires:
  VVec/1 -> Sum of Elements1/1
  Divide1/1 -> V/1
  Sum of Elements1/1 -> Divide1/1
  Num of Thermal Nodes/1 -> Divide1/2

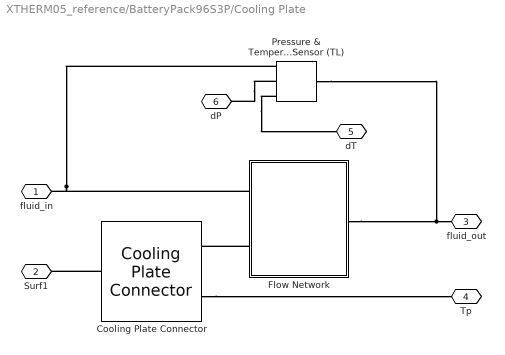
== system XTHERM05_reference/BatteryPack96S3P/Cooling Plate ==
  Cooling Plate Connector : coolingPlateThermal_lib/Cooling Plate Connector  plateTh=thkPlate m  plateThCond=thCondPlate W/(K*m)  plateDen=rhoPlate kg/m^3  plateCp=cpPlate J/(K*kg)  plateTemp_ini=initTempPlate K  plateDimX=plateDimX  plateDimY=plateDimY  numBattThermalNodes=numBattThermalNodes  dimensionThermalNodes=dimensionThermalNodes  locationThermalNodes=locationThermalNodes  numFluidElem=77  connfluidToPlateMat=[1 1;2 1;3 1;1 1;2 1;3 1;1 2;2 2;3 2;1 3;2 3;3 3;1 3;2 3;3 3;1 4;2 4;3 4;1 5;2 5;3 5;1 5;2 5;3 5;1 6;2 6;3 6;1 6;2 6;3 6;1 7;2 7;3 7;1 8;2 8;3 8;1 8;2 8;3 8;1 1;1 1;1 2;1 2;1 3;1 3;1 3;1 4;1 4;1 5;1 5;1 6;1 6;1 6;1 7;1 7;1 8;1 8;3 1;3 1;3 2;3 2;3 3;3 3;3 3;3 4;3 4;3 5;3 5;3 6;3 6;3 6;3 7;3 7;3 8;3 8;1 8;3 1]  plateConnectivity=simscape.battery.enum.thermal.coolingPlateConnectivity.singleSided
      settings: InternalSimscapePortConfiguration="{\"Bottom\":[],\"Left\":[{\"id\":\"Batt\",\"label\":\"B\",\"type\":\"foundation.thermal.thermal\"}],\"Right\":[{\"id\":\"Cool\",\"label\":\"H\",\"type\":\"foundation.thermal.thermal\"},{\"id\":\"plotPlateT\",\"label\":\"Tp\",\"type\":\"output\"}],\"Top\":[]}"
  Flow Network : Subsystem
      mask Display: image('CoolingPlateMaskIcon.png')
  Pressure & Temperature Sensor (TL) : fl_lib/Thermal Liquid/Sensors/Pressure & Temperature Sensor (TL)  reference=foundation.enum.MeasurementReference.difference  pressure=true  pressure_spec=foundation.enum.PressureMeasementSpec.Absolute  temperature=true
      settings: InternalSimscapePortConfiguration="{\"Bottom\":[{\"id\":\"T\",\"label\":\"T\",\"type\":\"output\"}],\"Left\":[{\"id\":\"A\",\"label\":\"A\",\"type\":\"foundation.thermal_liquid.thermal_liquid\"}],\"Right\":[{\"id\":\"B\",\"label\":\"B\",\"type\":\"foundation.thermal_liquid.thermal_liquid\"},{\"id\":\"P\",\"label\":\"P\",\"type\":\"output\"}],\"Top\":[]}"
  fluid_in : PMIOPort  Side=Left
  Surf1 : PMIOPort  Port=2  Side=Left
  fluid_out : PMIOPort  Port=3  Side=Right
  Tp : PMIOPort  Port=4  Side=Right
  dT : PMIOPort  Port=5  Side=Right
  dP : PMIOPort  Port=6  Side=Right
  connections:
  Pressure & Temperature Sensor (TL)/RConn2 -- dP/RConn1
  Pressure & Temperature Sensor (TL)/RConn3 -- dT/RConn1
  Cooling Plate Connector/RConn2 -- Tp/RConn1
  Cooling Plate Connector/LConn1 -- Surf1/RConn1
  Pressure & Temperature Sensor (TL)/LConn1 -- fluid_out/RConn1 -- Flow Network/RConn1
  Pressure & Temperature Sensor (TL)/RConn1 -- fluid_in/RConn1 -- Flow Network/LConn1
  Flow Network/LConn2 -- Cooling Plate Connector/RConn1

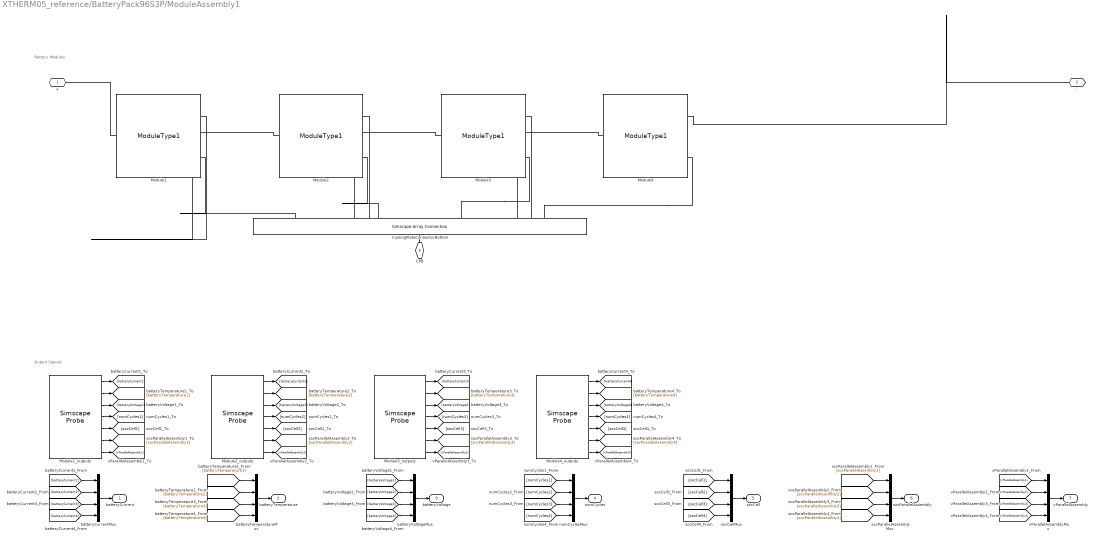
== system XTHERM05_reference/BatteryPack96S3P/ModuleAssembly1 ==
  note: Output Signals
  note: Battery Modules
  CoolingPlateConnectorBottom : SimscapeArrayConnection  Domain=foundation.thermal.thermal  Mode=Sized Elements
  Module{1..4} (4 alike) : BatteryPack96S3P_lib/Modules/ModuleType1  BatteryCapacityCell=78 A*hr  ExtrapolationMethodCell=simscape.enum.extrapolation.nearest  SOCBreakpointsCell=[0, .1, .25, .5, .75, .9, 1]  TemperatureBreakpointsCell=[278, 293, 313] K  OpenCircuitVoltageThermalCell=[3.49, 3.5, 3.51; 3.55, 3.57, 3.56; 3.62, 3.63, 3.64; 3.71, 3.71, 3.72; 3.91, 3.93, 3.94; 4.07, 4.08, 4.08; 4.19, 4.19, 4.19] V  VoltageRangeCell=[0, inf] V  ResistanceSOCBreakpointsCell=[0, .1, .25, .5, .75, .9, 1]  ResistanceTemperatureBreakpointsCell=[278, 293, 313] K  R0ThermalCell=[.0117, .0085, .009; .011, .0085, .009; .0114, .0087, .0092; .0107, .0082, .0088; .0107, .0083, .0091; .0113, .0085, .0089; .0116, .0085, .0089] Ohm  BatteryThermalMassCell=1083 J/K  NumThermalModelsCell=4  ThermalConductivityZCell=18 W/(K*m)  CrossSectionalAreaXYCell=0.003 m^2  HeightCell=0.2 m  CoolantResistance=1.2 K/W  P=3  S=8  SeriesGrouping=[4, 4]  ParallelGrouping=[1, 1]  socCell_specify=on  socCell_priority=High  socCell=[0.2 0.2]  socCell_nominal_specify=off  socCell_nominal_value=1  socCell_nominal_unit=1  batteryVoltage_specify=off  batteryVoltage_priority=None  batteryVoltage=repmat(0, 2, 1) V  batteryVoltage_nominal_specify=off  batteryVoltage_nominal_value=1  batteryVoltage_nominal_unit=V  batteryCurrent_specify=off  batteryCurrent_priority=None  batteryCurrent=repmat(0, 2, 1) A  batteryCurrent_nominal_specify=off  batteryCurrent_nominal_value=1  batteryCurrent_nominal_unit=A  numCycles_specify=off  numCycles_priority=High  numCycles=repmat(0, 2, 1)  numCycles_nominal_specify=off  numCycles_nominal_value=1  numCycles_nominal_unit=1  batteryTemperature_specify=on  batteryTemperature_priority=High  batteryTemperature=[initial_battery_temperature_K initial_battery_temperature_K] K  batteryTemperature_nominal_specify=off  batteryTemperature_nominal_value=1  batteryTemperature_nominal_unit=K  vParallelAssembly_specify=off  vParallelAssembly_priority=None  vParallelAssembly=repmat(0, 8, 1) V  vParallelAssembly_nominal_specify=off  vParallelAssembly_nominal_value=1  vParallelAssembly_nominal_unit=V  socParallelAssembly_specify=off  socParallelAssembly_priority=None  socParallelAssembly=repmat(1, 8, 1)  socParallelAssembly_nominal_specify=off  socParallelAssembly_nominal_value=1  socParallelAssembly_nominal_unit=1
      settings: InternalSimscapePortConfiguration="{\"Bottom\":[{\"id\":\"n\",\"label\":\"-\",\"type\":\"foundation.electrical.electrical\"},{\"id\":\"BottomExtClnt\",\"label\":\"CPB\",\"type\":\"foundation.thermal.thermal\"}],\"Left\":[],\"Right\":[],\"Top\":[{\"id\":\"p\",\"label\":\"+\",\"type\":\"foundation.electrical.electrical\"}]}"
  Module1_outputs : SimscapeProbe  BoundBlock=1291  Variables="{\"batteryCurrent\":{\"Probing\":\"ON\"},\"batteryTemperature\":{\"Probing\":\"ON\"},\"batteryVoltage\":{\"Probing\":\"ON\"},\"numCycles\":{\"Probing\":\"ON\"},\"socCell\":{\"Probing\":\"ON\"},\"socParallelAssembly\":{\"Probing\":\"ON\"},\"vParallelAssembly\":{\"Probing\":\"ON\"}}"
  Module2_outputs : SimscapeProbe  BoundBlock=1293  Variables="{\"batteryCurrent\":{\"Probing\":\"ON\"},\"batteryTemperature\":{\"Probing\":\"ON\"},\"batteryVoltage\":{\"Probing\":\"ON\"},\"numCycles\":{\"Probing\":\"ON\"},\"socCell\":{\"Probing\":\"ON\"},\"socParallelAssembly\":{\"Probing\":\"ON\"},\"vParallelAssembly\":{\"Probing\":\"ON\"}}"
  Module3_outputs : SimscapeProbe  BoundBlock=1295  Variables="{\"batteryCurrent\":{\"Probing\":\"ON\"},\"batteryTemperature\":{\"Probing\":\"ON\"},\"batteryVoltage\":{\"Probing\":\"ON\"},\"numCycles\":{\"Probing\":\"ON\"},\"socCell\":{\"Probing\":\"ON\"},\"socParallelAssembly\":{\"Probing\":\"ON\"},\"vParallelAssembly\":{\"Probing\":\"ON\"}}"
  Module4_outputs : SimscapeProbe  BoundBlock=1297  Variables="{\"batteryCurrent\":{\"Probing\":\"ON\"},\"batteryTemperature\":{\"Probing\":\"ON\"},\"batteryVoltage\":{\"Probing\":\"ON\"},\"numCycles\":{\"Probing\":\"ON\"},\"socCell\":{\"Probing\":\"ON\"},\"socParallelAssembly\":{\"Probing\":\"ON\"},\"vParallelAssembly\":{\"Probing\":\"ON\"}}"
  batteryCurrentMux : Mux
  batteryTemperatureMux : Mux
  batteryVoltageMux : Mux
  numCyclesMux : Mux
  socCellMux : Mux
  socParallelAssemblyMux : Mux
  vParallelAssemblyMux : Mux
  + : PMIOPort  Side=Left
  - : PMIOPort  Port=2  Side=Right
  CPB : PMIOPort  Port=3  Side=Right  ConnectionType=Connection: foundation.thermal.thermal
  batteryCurrent : Outport
  batteryTemperature : Outport  Port=2
  batteryVoltage : Outport  Port=3
  numCycles : Outport  Port=4
  socCell : Outport  Port=5
  socParallelAssembly : Outport  Port=6
  vParallelAssembly : Outport  Port=7
  wires:
  [vParallelAssembly4] -> vParallelAssemblyMux/4
  Module4_outputs/7 -> [vParallelAssembly4]
  [socParallelAssembly4] -> socParallelAssemblyMux/4
  Module4_outputs/6 -> [socParallelAssembly4]
  [socCell4] -> socCellMux/4
  Module4_outputs/5 -> [socCell4]
  [numCycles4] -> numCyclesMux/4
  Module4_outputs/4 -> [numCycles4]
  [batteryVoltage4] -> batteryVoltageMux/4
  Module4_outputs/3 -> [batteryVoltage4]
  [batteryTemperature4] -> batteryTemperatureMux/4
  Module4_outputs/2 -> [batteryTemperature4]
  [batteryCurrent4] -> batteryCurrentMux/4
  Module4_outputs/1 -> [batteryCurrent4]
  [vParallelAssembly3] -> vParallelAssemblyMux/3
  Module3_outputs/7 -> [vParallelAssembly3]
  [socParallelAssembly3] -> socParallelAssemblyMux/3
  Module3_outputs/6 -> [socParallelAssembly3]
  [socCell3] -> socCellMux/3
  Module3_outputs/5 -> [socCell3]
  [numCycles3] -> numCyclesMux/3
  Module3_outputs/4 -> [numCycles3]
  [batteryVoltage3] -> batteryVoltageMux/3
  Module3_outputs/3 -> [batteryVoltage3]
  [batteryTemperature3] -> batteryTemperatureMux/3
  Module3_outputs/2 -> [batteryTemperature3]
  [batteryCurrent3] -> batteryCurrentMux/3
  Module3_outputs/1 -> [batteryCurrent3]
  [vParallelAssembly2] -> vParallelAssemblyMux/2
  Module2_outputs/7 -> [vParallelAssembly2]
  [socParallelAssembly2] -> socParallelAssemblyMux/2
  Module2_outputs/6 -> [socParallelAssembly2]
  [socCell2] -> socCellMux/2
  Module2_outputs/5 -> [socCell2]
  [numCycles2] -> numCyclesMux/2
  Module2_outputs/4 -> [numCycles2]
  [batteryVoltage2] -> batteryVoltageMux/2
  Module2_outputs/3 -> [batteryVoltage2]
  [batteryTemperature2] -> batteryTemperatureMux/2
  Module2_outputs/2 -> [batteryTemperature2]
  [batteryCurrent2] -> batteryCurrentMux/2
  Module2_outputs/1 -> [batteryCurrent2]
  [vParallelAssembly1] -> vParallelAssemblyMux/1
  vParallelAssemblyMux/1 -> vParallelAssembly/1
  Module1_outputs/7 -> [vParallelAssembly1]
  [socParallelAssembly1] -> socParallelAssemblyMux/1
  socParallelAssemblyMux/1 -> socParallelAssembly/1
  Module1_outputs/6 -> [socParallelAssembly1]
  [socCell1] -> socCellMux/1
  socCellMux/1 -> socCell/1
  Module1_outputs/5 -> [socCell1]
  [numCycles1] -> numCyclesMux/1
  numCyclesMux/1 -> numCycles/1
  Module1_outputs/4 -> [numCycles1]
  [batteryVoltage1] -> batteryVoltageMux/1
  batteryVoltageMux/1 -> batteryVoltage/1
  Module1_outputs/3 -> [batteryVoltage1]
  [batteryTemperature1] -> batteryTemperatureMux/1
  batteryTemperatureMux/1 -> batteryTemperature/1
  Module1_outputs/2 -> [batteryTemperature1]
  [batteryCurrent1] -> batteryCurrentMux/1
  batteryCurrentMux/1 -> batteryCurrent/1
  Module1_outputs/1 -> [batteryCurrent1]
  connections:
  CoolingPlateConnectorBottom/RConn1 -- CPB/RConn1
  CoolingPlateConnectorBottom/LConn4 -- Module4/RConn2
  CoolingPlateConnectorBottom/LConn3 -- Module3/RConn2
  CoolingPlateConnectorBottom/LConn2 -- Module2/RConn2
  CoolingPlateConnectorBottom/LConn1 -- Module1/RConn2
  Module4/RConn1 -- -/RConn1
  Module1/LConn1 -- +/RConn1
  Module4/LConn1 -- Module3/RConn1
  Module3/LConn1 -- Module2/RConn1
  Module2/LConn1 -- Module1/RConn1
